simulink model "DSB-SC Modulation and demodulation"  (R2025a)
settings: Solver=VariableStepAuto  StartTime=0.0  StopTime=10.0  RelTol=1e-3
libraries: dspsrcs4 x3, dspfdesign x1
settings Model: Creator=Aman  LastModifiedBy=Aman

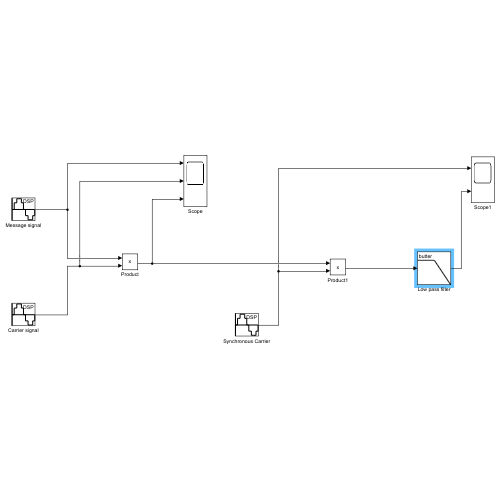
[thumbnail: Simulink's stored preview of the top-level diagram]
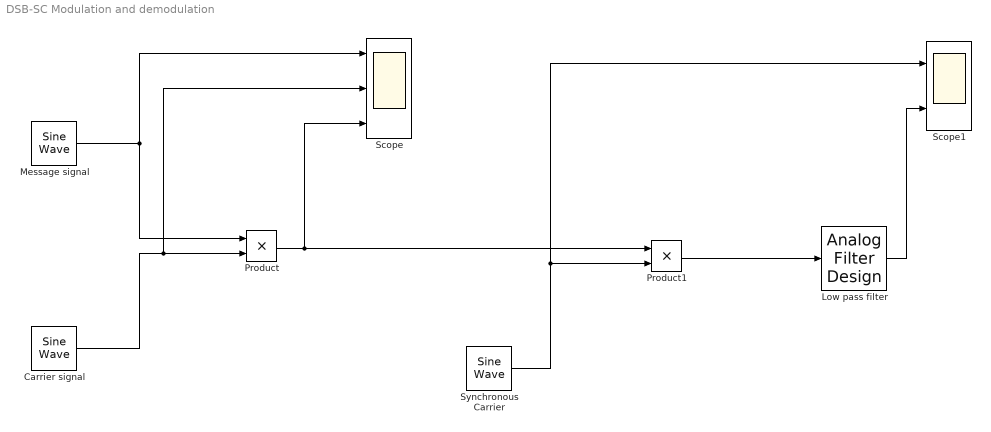
== system DSB-SC Modulation and demodulation ==
  Carrier signal : dspsrcs4/Sine Wave  Amplitude=2  Frequency=20  Phase=0  SampleMode=Discrete  OutComplex=Real  CompMethod=Trigonometric fcn  TableSize=Speed  SampleTime=1/1000  SamplesPerFrame=1  ResetState=Restart at time zero  OutputFrames=off  dataType=double  wordLen=16  udDataType=sfix(16)  fracBitsMode=Best precision  numFracBits=15  OutDataTypeStr=double  LastOutDataTypeStr=double
  Low pass filter : dspfdesign/Analog Filter Design  method=Butterworth  filttype=Lowpass  N=8  Wlo=2*pi*1  Whi=80  Rp=2  Rs=40
  Message signal : dspsrcs4/Sine Wave  Amplitude=1  Frequency=1  Phase=0  SampleMode=Discrete  OutComplex=Real  CompMethod=Trigonometric fcn  TableSize=Speed  SampleTime=1/1000  SamplesPerFrame=1  ResetState=Restart at time zero  OutputFrames=off  dataType=double  wordLen=16  udDataType=sfix(16)  fracBitsMode=Best precision  numFracBits=15  OutDataTypeStr=double  LastOutDataTypeStr=double
  Product : Product
  Product1 : Product
  Scope : Scope  NumInputPorts=3
      settings: ActiveDisplayYMinimum=-5.1269230769230774  ActiveDisplayYMaximum=1.1230769230769231
  Scope1 : Scope  NumInputPorts=2
      settings: ActiveDisplayYMinimum=-2.1259445954959761  ActiveDisplayYMaximum=2.2469428494240962
  Synchronous Carrier : dspsrcs4/Sine Wave  Amplitude=2  Frequency=20  Phase=0  SampleMode=Discrete  OutComplex=Real  CompMethod=Trigonometric fcn  TableSize=Speed  SampleTime=1/1000  SamplesPerFrame=1  ResetState=Restart at time zero  OutputFrames=off  dataType=double  wordLen=16  udDataType=sfix(16)  fracBitsMode=Best precision  numFracBits=15  OutDataTypeStr=double  LastOutDataTypeStr=double
  wires:
  Message signal/1 -> Product/1, Scope/1
  Carrier signal/1 -> Scope/2, Product/2
  Product/1 -> Scope/3, Product1/1
  Synchronous Carrier/1 -> Scope1/1, Product1/2
  Product1/1 -> Low pass filter/1
  Low pass filter/1 -> Scope1/2
